simulink model "DRL_MPC_MATLAB"  (R2025a)
settings: Solver=FixedStepDiscrete  StartTime=0.0  StopTime=20  FixedStep=0.0005  RelTol=1e-3
PostLoadFcn:
  | addpath(fileparts(fileparts(get_param('DRL_MPC_MATLAB','FileName'))));setup_matlab_mpc;
undefined symbols (not defined in the file): controller_mode, mpc_initial_control_result, steering_interface_test, steering_test_deg
libraries: Solver_SF x1, rllib x1
settings Model: Creator=fengchengmin  LastModifiedBy=fengchengmin

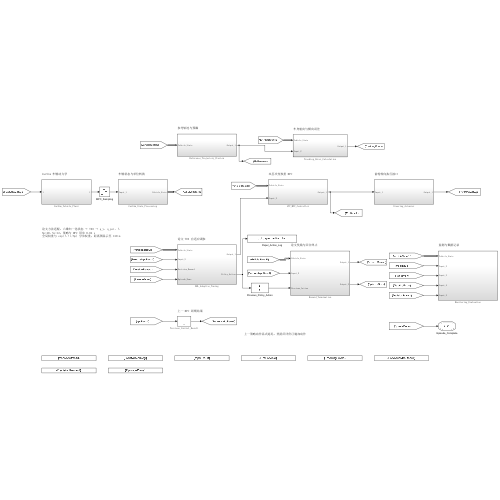
[thumbnail: Simulink's stored preview of the top-level diagram]
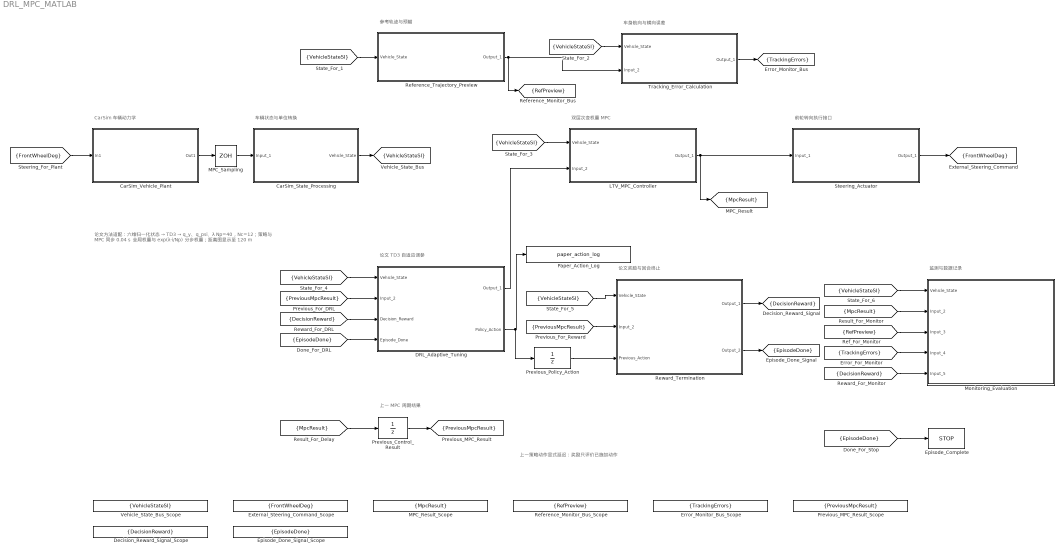
== system DRL_MPC_MATLAB ==
  note: 论文方法适配：六维归一化状态 → TD3 → q_y、q_psi、λ
      | Np=40，Nc=12；策略与 MPC 同步 0.04 s
      | 全局权重与 exp(λ·i/Np) 分步权重；距离图显示至 120 m
  note: 上一策略动作显式延迟：奖励只评价已施加动作
  note: CarSim 车辆动力学
  note: 车辆状态与单位转换
  note: 参考轨迹与预瞄
  note: 车身航向与横向误差
  note: 双层次变权重 MPC
  note: 论文 TD3 自适应调参
  note: 前轮转向执行接口
  note: 监测与数据记录
  note: 论文奖励与回合终止
  note: 上一 MPC 周期结果
  CarSim_State_Processing : Subsystem
  CarSim_Vehicle_Plant : Subsystem
  DRL_Adaptive_Tuning : Subsystem
  Decision_Reward_Signal_Scope : GotoTagVisibility  GotoTag=DecisionReward
  Episode_Complete : Stop
  Episode_Done_Signal_Scope : GotoTagVisibility  GotoTag=EpisodeDone
  Error_Monitor_Bus_Scope : GotoTagVisibility  GotoTag=TrackingErrors
  External_Steering_Command_Scope : GotoTagVisibility  GotoTag=FrontWheelDeg
  LTV_MPC_Controller : Subsystem
  MPC_Result_Scope : GotoTagVisibility  GotoTag=MpcResult
  MPC_Sampling : ZeroOrderHold  SampleTime=0.04
  Monitoring_Evaluation : Subsystem
  Paper_Action_Log : ToWorkspace  VariableName=paper_action_log  SaveFormat=Timeseries  SampleTime=-1
  Previous_Control_Result : UnitDelay  InitialCondition=mpc_initial_control_result  SampleTime=0.04  HasFrameUpgradeWarning=on
  Previous_MPC_Result_Scope : GotoTagVisibility  GotoTag=PreviousMpcResult
  Previous_Policy_Action : UnitDelay  InitialCondition=zeros(3,1)  SampleTime=.04  HasFrameUpgradeWarning=on
  Reference_Monitor_Bus_Scope : GotoTagVisibility  GotoTag=RefPreview
  Reference_Trajectory_Preview : Subsystem
  Reward_Termination : Subsystem
  Steering_Actuator : Subsystem
  Tracking_Error_Calculation : Subsystem
  Vehicle_State_Bus_Scope : GotoTagVisibility  GotoTag=VehicleStateSI
  tag scope: DecisionReward=scoped, EpisodeDone=scoped, FrontWheelDeg=scoped, MpcResult=scoped, PreviousMpcResult=scoped, RefPreview=scoped, TrackingErrors=scoped, VehicleStateSI=scoped
  wires:
  Tracking_Error_Calculation/1(Output_1) -> [TrackingErrors]
  Previous_Control_Result/1 -> [PreviousMpcResult]
  Reward_Termination/1(Output_1) -> [DecisionReward]
  Reward_Termination/2(Output_2) -> [EpisodeDone]
  [RefPreview] -> Monitoring_Evaluation/3(Input_3)
  [TrackingErrors] -> Monitoring_Evaluation/4(Input_4)
  [DecisionReward] -> Monitoring_Evaluation/5(Input_5)
  [EpisodeDone] -> Episode_Complete/1
  Steering_Actuator/1(Output_1) -> [FrontWheelDeg]
  [VehicleStateSI] -> LTV_MPC_Controller/1(Vehicle_State)
  [VehicleStateSI] -> Monitoring_Evaluation/1(Vehicle_State)
  CarSim_State_Processing/1(Vehicle_State) -> [VehicleStateSI]
  [FrontWheelDeg] -> CarSim_Vehicle_Plant/1(In1)
  [MpcResult] -> Previous_Control_Result/1
  [MpcResult] -> Monitoring_Evaluation/2(Input_2)
  LTV_MPC_Controller/1(Output_1) -> [MpcResult], Steering_Actuator/1(Input_1)
  MPC_Sampling/1 -> CarSim_State_Processing/1(Input_1)
  CarSim_Vehicle_Plant/1(Out1) -> MPC_Sampling/1
  [PreviousMpcResult] -> Reward_Termination/2(Input_2)
  Reference_Trajectory_Preview/1(Output_1) -> [RefPreview], Tracking_Error_Calculation/2(Input_2)
  [PreviousMpcResult] -> DRL_Adaptive_Tuning/2(Input_2)
  [DecisionReward] -> DRL_Adaptive_Tuning/3(Decision_Reward)
  [EpisodeDone] -> DRL_Adaptive_Tuning/4(Episode_Done)
  [VehicleStateSI] -> Reference_Trajectory_Preview/1(Vehicle_State)
  [VehicleStateSI] -> Tracking_Error_Calculation/1(Vehicle_State)
  [VehicleStateSI] -> DRL_Adaptive_Tuning/1(Vehicle_State)
  [VehicleStateSI] -> Reward_Termination/1(Vehicle_State)
  DRL_Adaptive_Tuning/1(Output_1) -> LTV_MPC_Controller/2(Input_2)
  Previous_Policy_Action/1 -> Reward_Termination/3(Previous_Action)
  DRL_Adaptive_Tuning/2(Policy_Action) -> Previous_Policy_Action/1, Paper_Action_Log/1

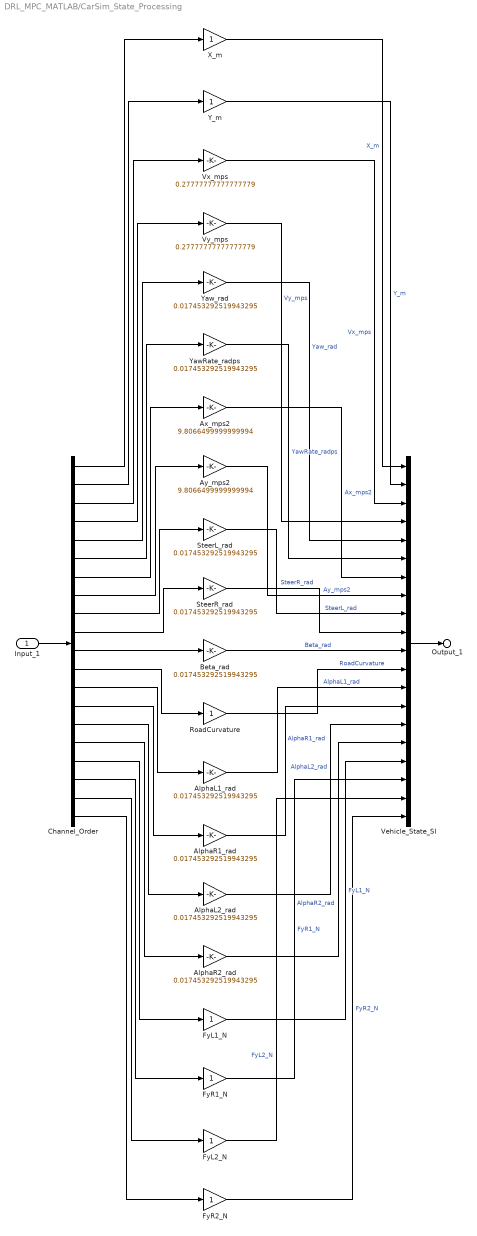
== system DRL_MPC_MATLAB/CarSim_State_Processing ==
  Input_1 : Inport
  AlphaL1_rad : Gain  Gain=0.017453292519943295
  AlphaL2_rad : Gain  Gain=0.017453292519943295
  AlphaR1_rad : Gain  Gain=0.017453292519943295
  AlphaR2_rad : Gain  Gain=0.017453292519943295
  Ax_mps2 : Gain  Gain=9.8066499999999994
  Ay_mps2 : Gain  Gain=9.8066499999999994
  Beta_rad : Gain  Gain=0.017453292519943295
  Channel_Order : Demux  Outputs=20
  FyL1_N : Gain
  FyL2_N : Gain
  FyR1_N : Gain
  FyR2_N : Gain
  RoadCurvature : Gain
  SteerL_rad : Gain  Gain=0.017453292519943295
  SteerR_rad : Gain  Gain=0.017453292519943295
  Vehicle_State_SI : BusCreator  Inputs=20
  Vx_mps : Gain  Gain=0.27777777777777779
  Vy_mps : Gain  Gain=0.27777777777777779
  X_m : Gain
  Y_m : Gain
  YawRate_radps : Gain  Gain=0.017453292519943295
  Yaw_rad : Gain  Gain=0.017453292519943295
  Output_1 : Outport  PortName=Vehicle_State
  wires:
  Vehicle_State_SI/1 -> Output_1/1
  FyR2_N/1 -> Vehicle_State_SI/20  "FyR2_N"
  Channel_Order/20 -> FyR2_N/1
  FyL2_N/1 -> Vehicle_State_SI/19  "FyL2_N"
  Channel_Order/19 -> FyL2_N/1
  FyR1_N/1 -> Vehicle_State_SI/18  "FyR1_N"
  Channel_Order/18 -> FyR1_N/1
  FyL1_N/1 -> Vehicle_State_SI/17  "FyL1_N"
  Channel_Order/17 -> FyL1_N/1
  AlphaR2_rad/1 -> Vehicle_State_SI/16  "AlphaR2_rad"
  Channel_Order/15 -> AlphaL2_rad/1
  Channel_Order/16 -> AlphaR2_rad/1
  AlphaL2_rad/1 -> Vehicle_State_SI/15  "AlphaL2_rad"
  AlphaR1_rad/1 -> Vehicle_State_SI/14  "AlphaR1_rad"
  Channel_Order/14 -> AlphaR1_rad/1
  AlphaL1_rad/1 -> Vehicle_State_SI/13  "AlphaL1_rad"
  Channel_Order/13 -> AlphaL1_rad/1
  RoadCurvature/1 -> Vehicle_State_SI/12  "RoadCurvature"
  Channel_Order/12 -> RoadCurvature/1
  Beta_rad/1 -> Vehicle_State_SI/11  "Beta_rad"
  Channel_Order/11 -> Beta_rad/1
  SteerR_rad/1 -> Vehicle_State_SI/10  "SteerR_rad"
  Channel_Order/10 -> SteerR_rad/1
  SteerL_rad/1 -> Vehicle_State_SI/9  "SteerL_rad"
  Channel_Order/9 -> SteerL_rad/1
  Ay_mps2/1 -> Vehicle_State_SI/8  "Ay_mps2"
  Channel_Order/8 -> Ay_mps2/1
  Ax_mps2/1 -> Vehicle_State_SI/7  "Ax_mps2"
  Channel_Order/7 -> Ax_mps2/1
  YawRate_radps/1 -> Vehicle_State_SI/6  "YawRate_radps"
  Channel_Order/6 -> YawRate_radps/1
  Yaw_rad/1 -> Vehicle_State_SI/5  "Yaw_rad"
  Channel_Order/5 -> Yaw_rad/1
  Vy_mps/1 -> Vehicle_State_SI/4  "Vy_mps"
  Channel_Order/4 -> Vy_mps/1
  Vx_mps/1 -> Vehicle_State_SI/3  "Vx_mps"
  Channel_Order/3 -> Vx_mps/1
  Y_m/1 -> Vehicle_State_SI/2  "Y_m"
  Channel_Order/2 -> Y_m/1
  X_m/1 -> Vehicle_State_SI/1  "X_m"
  Channel_Order/1 -> X_m/1
  Input_1/1 -> Channel_Order/1

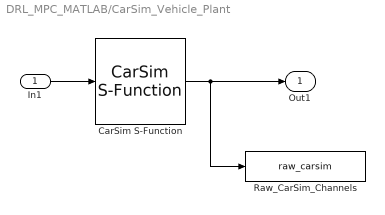
== system DRL_MPC_MATLAB/CarSim_Vehicle_Plant ==
  In1 : Inport
  CarSim S-Function : Solver_SF/CarSim S-Function  Priority=1  SIMFILE=C:\Users\fengchengmin\Desktop\JQRKZ\DRL-MPC\matlab\carsim\case\simfile.sim  Run_RTs=off  vs_state_ind=Run  StopMode_ind=Vehicle Model
  Raw_CarSim_Channels : ToWorkspace  VariableName=raw_carsim  SaveFormat=Timeseries  SampleTime=-1
  Out1 : Outport
  wires:
  CarSim S-Function/1 -> Out1/1, Raw_CarSim_Channels/1
  In1/1 -> CarSim S-Function/1

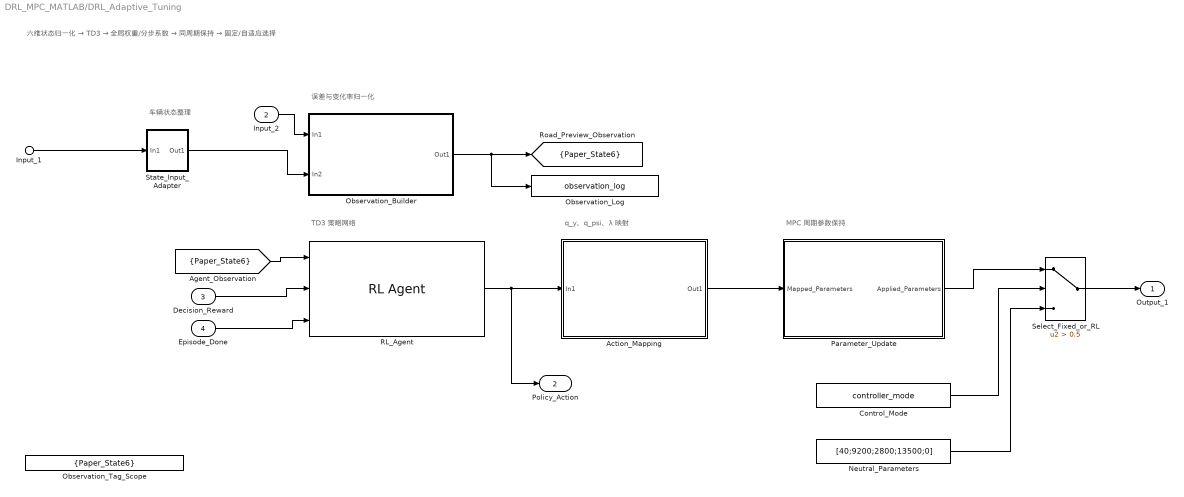
== system DRL_MPC_MATLAB/DRL_Adaptive_Tuning ==
  note: 六维状态归一化 → TD3 → 全局权重/分步系数 → 同周期保持 → 固定/自适应选择
  note: 车辆状态整理
  note: 误差与变化率归一化
  note: TD3 策略网络
  note: q_y、q_psi、λ 映射
  note: MPC 周期参数保持
  Input_1 : Inport  PortName=Vehicle_State
  Input_2 : Inport  Port=2
  Decision_Reward : Inport  Port=3
  Episode_Done : Inport  Port=4
  Action_Mapping : Subsystem
  Control_Mode : Constant  Value=controller_mode
  Neutral_Parameters : Constant  Value=[40;9200;2800;13500;0]
  Observation_Builder : Subsystem
  Observation_Log : ToWorkspace  VariableName=observation_log  SaveFormat=Timeseries  SampleTime=-1
  Observation_Tag_Scope : GotoTagVisibility  GotoTag=Paper_State6
  Parameter_Update : Subsystem
  RL_Agent : rllib/RL Agent  Agent=agent  ExternalActionAsInput=off  ProvideLastAction=off  ProvideCumRwd=off  TreatAsDirectFeedthrough=on  UseStrictObservationDataTypes=off
  Select_Fixed_or_RL : Switch  Criteria=u2 > Threshold  Threshold=0.5  SaturateOnIntegerOverflow=off  InputSameDT=off
  State_Input_Adapter : Subsystem
  Output_1 : Outport
  Policy_Action : Outport  Port=2
  tag scope: Paper_State6=scoped
  wires:
  Action_Mapping/1(Out1) -> Parameter_Update/1(Mapped_Parameters)
  Episode_Done/1 -> RL_Agent/3
  Decision_Reward/1 -> RL_Agent/2
  Input_2/1 -> Observation_Builder/1(In1)
  RL_Agent/1 -> Action_Mapping/1(In1), Policy_Action/1
  [Paper_State6] -> RL_Agent/1
  Select_Fixed_or_RL/1 -> Output_1/1
  Control_Mode/1 -> Select_Fixed_or_RL/2
  Neutral_Parameters/1 -> Select_Fixed_or_RL/3
  Observation_Builder/1(Out1) -> Observation_Log/1, [Paper_State6]
  Parameter_Update/1(Applied_Parameters) -> Select_Fixed_or_RL/1
  State_Input_Adapter/1(Out1) -> Observation_Builder/2(In2)
  Input_1/1 -> State_Input_Adapter/1(In1)

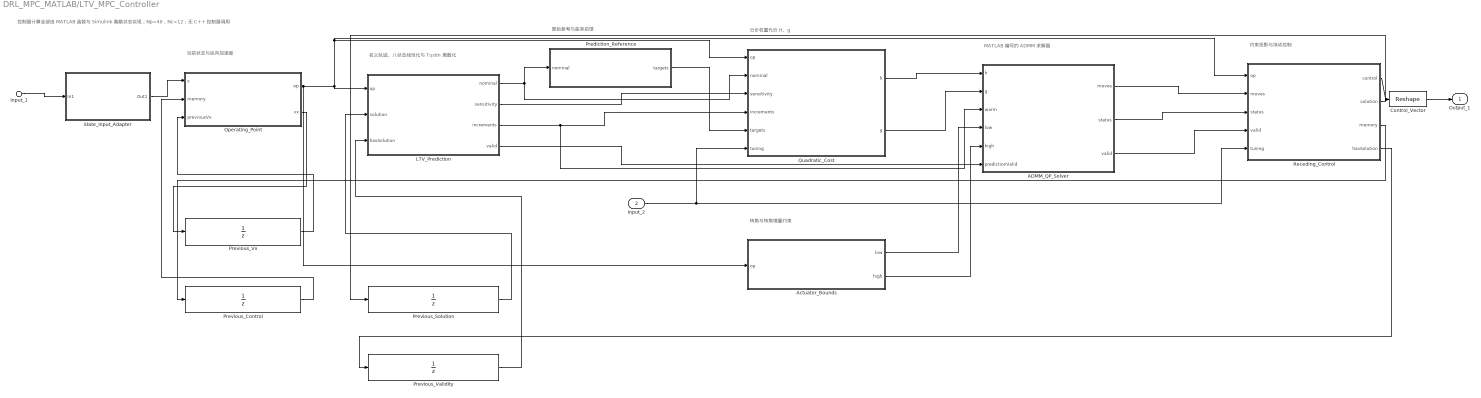
== system DRL_MPC_MATLAB/LTV_MPC_Controller ==
  note: 当前状态与纵向加速度
  note: 名义轨迹、八状态线性化与 Tustin 离散化
  note: 原始参考与曲率前馈
  note: 分步权重代价 H、g
  note: 转角与转角增量约束
  note: MATLAB 编写的 ADMM 求解器
  note: 约束投影与滚动控制
  note: 控制器计算全部由 MATLAB 函数与 Simulink 离散状态实现；Np=40，Nc=12；无 C++ 控制器调用
  Input_1 : Inport  PortName=Vehicle_State
  Input_2 : Inport  Port=2
  ADMM_QP_Solver : MATLAB Function  TreatAsAtomicUnit=on
  Actuator_Bounds : MATLAB Function  TreatAsAtomicUnit=on
  Control_Vector : Reshape
  LTV_Prediction : MATLAB Function  TreatAsAtomicUnit=on
  Operating_Point : MATLAB Function  TreatAsAtomicUnit=on
  Prediction_Reference : MATLAB Function  TreatAsAtomicUnit=on
  Previous_Control : UnitDelay  InitialCondition=[0;0]  SampleTime=.04  HasFrameUpgradeWarning=on
  Previous_Solution : UnitDelay  InitialCondition=zeros(12,1)  SampleTime=.04  HasFrameUpgradeWarning=on
  Previous_Validity : UnitDelay  InitialCondition=false  SampleTime=.04  HasFrameUpgradeWarning=on
  Previous_Vx : UnitDelay  InitialCondition=NaN  SampleTime=.04  HasFrameUpgradeWarning=on
  Quadratic_Cost : MATLAB Function  TreatAsAtomicUnit=on
  Receding_Control : MATLAB Function  TreatAsAtomicUnit=on
  State_Input_Adapter : Subsystem
  Output_1 : Outport
  wires:
  Input_1/1 -> State_Input_Adapter/1(In1)
  State_Input_Adapter/1(Out1) -> Operating_Point/1(s)
  Previous_Control/1 -> Operating_Point/2(memory)
  Previous_Vx/1 -> Operating_Point/3(previousVx)
  Operating_Point/2(vx) -> Previous_Vx/1
  Operating_Point/1(op) -> Quadratic_Cost/1(op), Receding_Control/1(op), LTV_Prediction/1(op), Actuator_Bounds/1(op)
  Previous_Solution/1 -> LTV_Prediction/2(solution)
  Previous_Validity/1 -> LTV_Prediction/3(hasSolution)
  LTV_Prediction/1(nominal) -> Prediction_Reference/1(nominal), Quadratic_Cost/2(nominal)
  LTV_Prediction/2(sensitivity) -> Quadratic_Cost/3(sensitivity)
  LTV_Prediction/3(increments) -> Quadratic_Cost/4(increments), ADMM_QP_Solver/3(warm)
  Prediction_Reference/1(targets) -> Quadratic_Cost/5(targets)
  Input_2/1 -> Quadratic_Cost/6(tuning), Receding_Control/5(tuning)
  Quadratic_Cost/1(h) -> ADMM_QP_Solver/1(h)
  Quadratic_Cost/2(g) -> ADMM_QP_Solver/2(g)
  Actuator_Bounds/1(low) -> ADMM_QP_Solver/4(low)
  Actuator_Bounds/2(high) -> ADMM_QP_Solver/5(high)
  LTV_Prediction/4(valid) -> ADMM_QP_Solver/6(predictionValid)
  ADMM_QP_Solver/1(moves) -> Receding_Control/2(moves)
  ADMM_QP_Solver/2(status) -> Receding_Control/3(status)
  ADMM_QP_Solver/3(valid) -> Receding_Control/4(valid)
  Receding_Control/1(control) -> Control_Vector/1
  Control_Vector/1 -> Output_1/1
  Receding_Control/2(solution) -> Previous_Solution/1
  Receding_Control/3(memory) -> Previous_Control/1
  Receding_Control/4(hasSolution) -> Previous_Validity/1

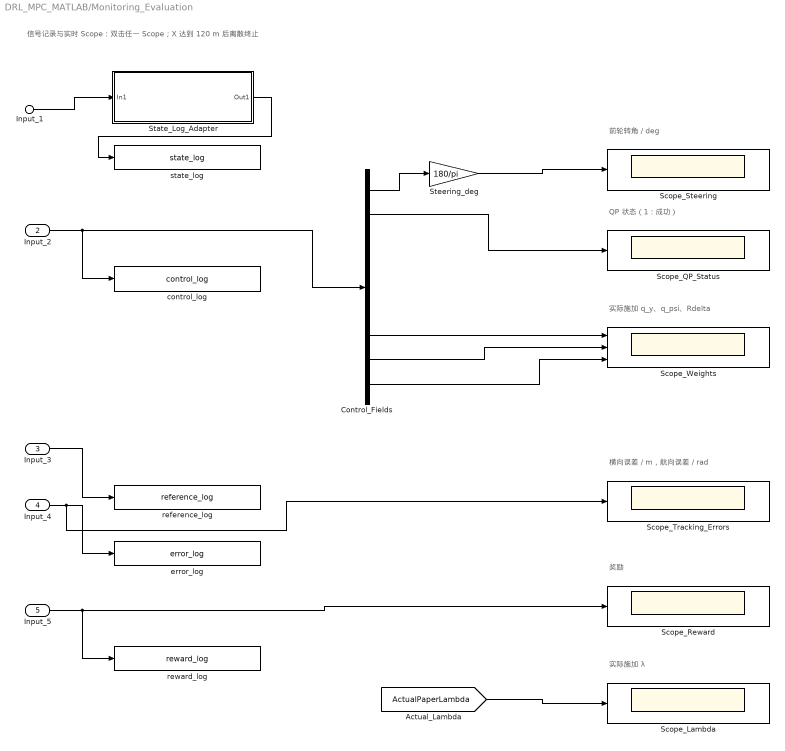
== system DRL_MPC_MATLAB/Monitoring_Evaluation ==
  note: 前轮转角 / deg
  note: QP 状态（1：成功）
  note: 实际施加 q_y、q_psi、Rdelta
  note: 横向误差 / m，航向误差 / rad
  note: 奖励
  note: 实际施加 λ
  note: 信号记录与实时 Scope：双击任一 Scope；X 达到 120 m 后离散终止
  Input_1 : Inport  PortName=Vehicle_State
  Input_2 : Inport  Port=2
  Input_3 : Inport  Port=3
  Input_4 : Inport  Port=4
  Input_5 : Inport  Port=5
  Control_Fields : Demux  Outputs=9
  Scope_Lambda : Scope
      settings: TimeSpan=8
  Scope_QP_Status : Scope
      settings: TimeSpan=8
  Scope_Reward : Scope
      settings: TimeSpan=8
  Scope_Steering : Scope
      settings: TimeSpan=8
  Scope_Tracking_Errors : Scope
      settings: TimeSpan=8
  Scope_Weights : Scope  NumInputPorts=3
      settings: TimeSpan=8
  State_Log_Adapter : Subsystem
  Steering_deg : Gain  Gain=180/pi
  control_log : ToWorkspace  VariableName=control_log  SaveFormat=Timeseries  SampleTime=-1
  error_log : ToWorkspace  VariableName=error_log  SaveFormat=Timeseries  SampleTime=-1
  reference_log : ToWorkspace  VariableName=reference_log  SaveFormat=Timeseries  SampleTime=-1
  reward_log : ToWorkspace  VariableName=reward_log  SaveFormat=Timeseries  SampleTime=-1
  state_log : ToWorkspace  VariableName=state_log  SaveFormat=Timeseries  SampleTime=-1
  wires:
  Input_5/1 -> reward_log/1, Scope_Reward/1
  Input_4/1 -> error_log/1, Scope_Tracking_Errors/1
  Input_3/1 -> reference_log/1
  Input_2/1 -> control_log/1, Control_Fields/1
  Control_Fields/1 -> Steering_deg/1
  Steering_deg/1 -> Scope_Steering/1
  Control_Fields/7 -> Scope_Weights/1
  Control_Fields/8 -> Scope_Weights/2
  Control_Fields/9 -> Scope_Weights/3
  Control_Fields/2 -> Scope_QP_Status/1
  [ActualPaperLambda] -> Scope_Lambda/1
  Input_1/1 -> State_Log_Adapter/1(In1)
  State_Log_Adapter/1(Out1) -> state_log/1

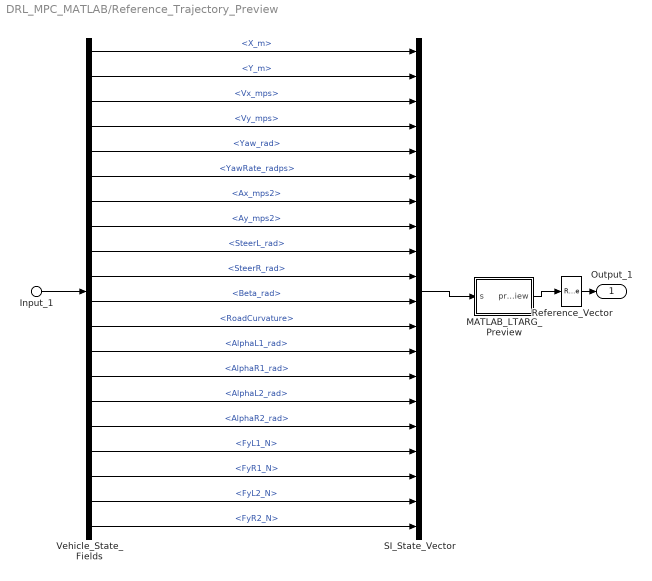
== system DRL_MPC_MATLAB/Reference_Trajectory_Preview ==
  Input_1 : Inport  PortName=Vehicle_State
  MATLAB_LTARG_Preview : MATLAB Function  TreatAsAtomicUnit=on
  Reference_Vector : Reshape
  SI_State_Vector : Mux  Inputs=20
  Vehicle_State_Fields : BusSelector  OutputSignals=X_m,Y_m,Vx_mps,Vy_mps,Yaw_rad,YawRate_radps,Ax_mps2,Ay_mps2,SteerL_rad,SteerR_rad,Beta_rad,RoadCurvature,AlphaL1_rad,AlphaR1_rad,AlphaL2_rad,AlphaR2_rad,FyL1_N,FyR1_N,FyL2_N,FyR2_N
  Output_1 : Outport
  wires:
  Input_1/1 -> Vehicle_State_Fields/1
  Vehicle_State_Fields/4 -> SI_State_Vector/4  "<Vy_mps>"
  Vehicle_State_Fields/5 -> SI_State_Vector/5  "<Yaw_rad>"
  Vehicle_State_Fields/20 -> SI_State_Vector/20  "<FyR2_N>"
  Vehicle_State_Fields/19 -> SI_State_Vector/19  "<FyL2_N>"
  Vehicle_State_Fields/18 -> SI_State_Vector/18  "<FyR1_N>"
  Vehicle_State_Fields/17 -> SI_State_Vector/17  "<FyL1_N>"
  Vehicle_State_Fields/16 -> SI_State_Vector/16  "<AlphaR2_rad>"
  Vehicle_State_Fields/15 -> SI_State_Vector/15  "<AlphaL2_rad>"
  Vehicle_State_Fields/14 -> SI_State_Vector/14  "<AlphaR1_rad>"
  Vehicle_State_Fields/13 -> SI_State_Vector/13  "<AlphaL1_rad>"
  Vehicle_State_Fields/12 -> SI_State_Vector/12  "<RoadCurvature>"
  Vehicle_State_Fields/11 -> SI_State_Vector/11  "<Beta_rad>"
  Vehicle_State_Fields/10 -> SI_State_Vector/10  "<SteerR_rad>"
  Vehicle_State_Fields/9 -> SI_State_Vector/9  "<SteerL_rad>"
  Vehicle_State_Fields/8 -> SI_State_Vector/8  "<Ay_mps2>"
  Vehicle_State_Fields/7 -> SI_State_Vector/7  "<Ax_mps2>"
  Vehicle_State_Fields/6 -> SI_State_Vector/6  "<YawRate_radps>"
  Vehicle_State_Fields/3 -> SI_State_Vector/3  "<Vx_mps>"
  Vehicle_State_Fields/2 -> SI_State_Vector/2  "<Y_m>"
  Vehicle_State_Fields/1 -> SI_State_Vector/1  "<X_m>"
  SI_State_Vector/1 -> MATLAB_LTARG_Preview/1(s)
  MATLAB_LTARG_Preview/1(preview) -> Reference_Vector/1
  Reference_Vector/1 -> Output_1/1

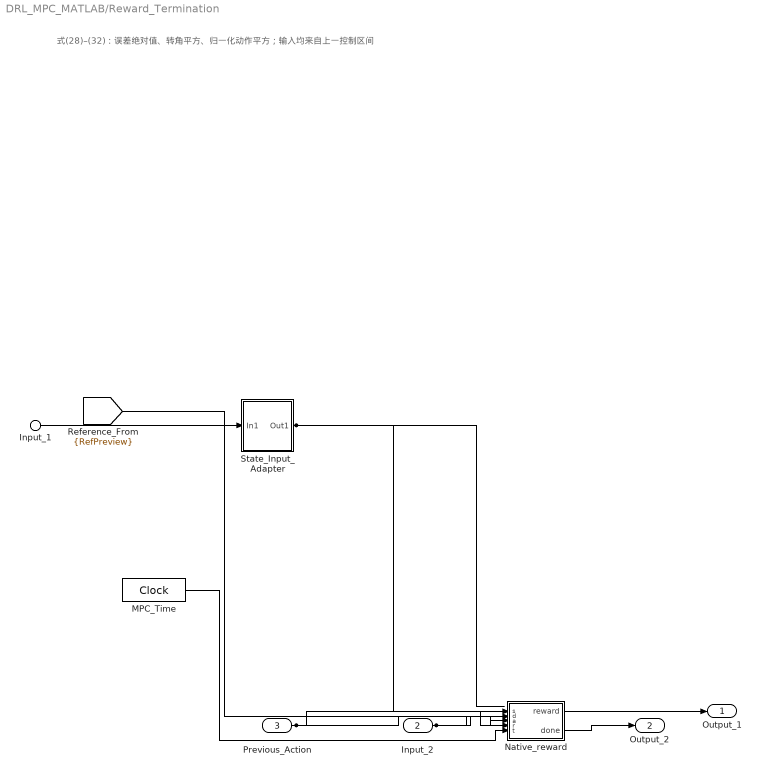
== system DRL_MPC_MATLAB/Reward_Termination ==
  note: 式(28)–(32)：误差绝对值、转角平方、归一化动作平方；输入均来自上一控制区间
  Input_1 : Inport  PortName=Vehicle_State
  Input_2 : Inport  Port=2
  Previous_Action : Inport  Port=3
  MPC_Time : DigitalClock  SampleTime=.04
  Native_reward : MATLAB Function  TreatAsAtomicUnit=on
  State_Input_Adapter : Subsystem
  Output_1 : Outport
  Output_2 : Outport  Port=2
  wires:
  Input_2/1 -> Native_reward/2(d)
  Previous_Action/1 -> Native_reward/3(a)
  State_Input_Adapter/1(Out1) -> Native_reward/1(s)
  Input_1/1 -> State_Input_Adapter/1(In1)
  [RefPreview] -> Native_reward/4(r)
  MPC_Time/1 -> Native_reward/5(t)
  Native_reward/1(reward) -> Output_1/1
  Native_reward/2(done) -> Output_2/1

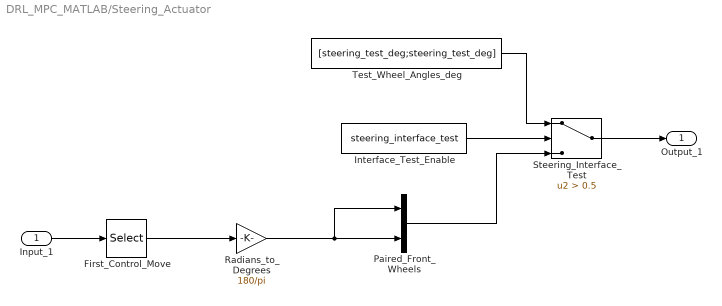
== system DRL_MPC_MATLAB/Steering_Actuator ==
  Input_1 : Inport
  First_Control_Move : Selector  InputPortWidth=9  IndexOptions=Index vector (dialog)  Indices=1  OutputSizes=1
  Interface_Test_Enable : Constant  Value=steering_interface_test
  Paired_Front_Wheels : Mux  Inputs=2
  Radians_to_Degrees : Gain  Gain=180/pi
  Steering_Interface_Test : Switch  Criteria=u2 > Threshold  Threshold=0.5  SaturateOnIntegerOverflow=off  InputSameDT=off
  Test_Wheel_Angles_deg : Constant  Value=[steering_test_deg;steering_test_deg]
  Output_1 : Outport
  wires:
  Paired_Front_Wheels/1 -> Steering_Interface_Test/3
  Test_Wheel_Angles_deg/1 -> Steering_Interface_Test/1
  Interface_Test_Enable/1 -> Steering_Interface_Test/2
  Steering_Interface_Test/1 -> Output_1/1
  Radians_to_Degrees/1 -> Paired_Front_Wheels/2, Paired_Front_Wheels/1
  First_Control_Move/1 -> Radians_to_Degrees/1
  Input_1/1 -> First_Control_Move/1

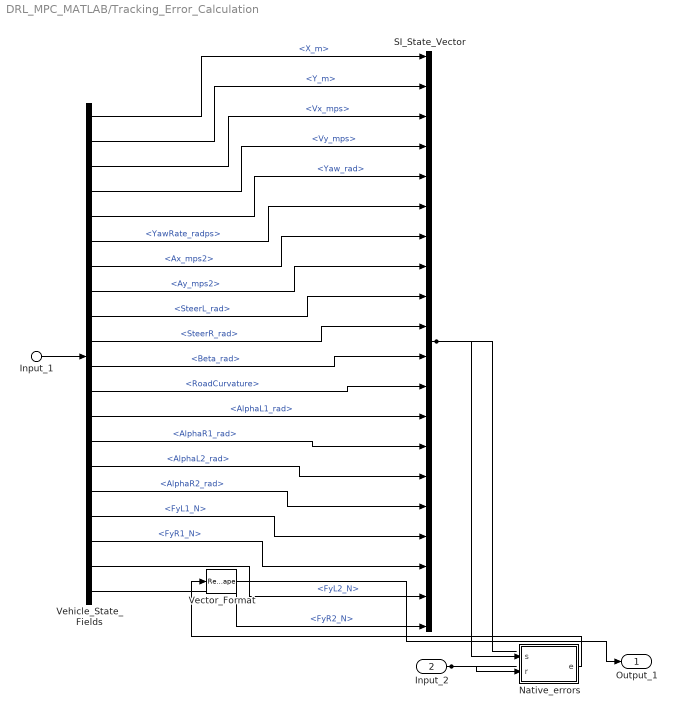
== system DRL_MPC_MATLAB/Tracking_Error_Calculation ==
  Input_1 : Inport  PortName=Vehicle_State
  Input_2 : Inport  Port=2
  Native_errors : MATLAB Function  TreatAsAtomicUnit=on
  SI_State_Vector : Mux  Inputs=20
  Vector_Format : Reshape
  Vehicle_State_Fields : BusSelector  OutputSignals=X_m,Y_m,Vx_mps,Vy_mps,Yaw_rad,YawRate_radps,Ax_mps2,Ay_mps2,SteerL_rad,SteerR_rad,Beta_rad,RoadCurvature,AlphaL1_rad,AlphaR1_rad,AlphaL2_rad,AlphaR2_rad,FyL1_N,FyR1_N,FyL2_N,FyR2_N
  Output_1 : Outport
  wires:
  Input_1/1 -> Vehicle_State_Fields/1
  Input_2/1 -> Native_errors/2(r)
  Vehicle_State_Fields/17 -> SI_State_Vector/17  "<FyL1_N>"
  SI_State_Vector/1 -> Native_errors/1(s)
  Vehicle_State_Fields/4 -> SI_State_Vector/4  "<Vy_mps>"
  Vehicle_State_Fields/5 -> SI_State_Vector/5  "<Yaw_rad>"
  Vehicle_State_Fields/20 -> SI_State_Vector/20  "<FyR2_N>"
  Vehicle_State_Fields/19 -> SI_State_Vector/19  "<FyL2_N>"
  Vehicle_State_Fields/18 -> SI_State_Vector/18  "<FyR1_N>"
  Vehicle_State_Fields/16 -> SI_State_Vector/16  "<AlphaR2_rad>"
  Vehicle_State_Fields/15 -> SI_State_Vector/15  "<AlphaL2_rad>"
  Vehicle_State_Fields/14 -> SI_State_Vector/14  "<AlphaR1_rad>"
  Vehicle_State_Fields/13 -> SI_State_Vector/13  "<AlphaL1_rad>"
  Vehicle_State_Fields/12 -> SI_State_Vector/12  "<RoadCurvature>"
  Vehicle_State_Fields/11 -> SI_State_Vector/11  "<Beta_rad>"
  Vehicle_State_Fields/10 -> SI_State_Vector/10  "<SteerR_rad>"
  Vehicle_State_Fields/9 -> SI_State_Vector/9  "<SteerL_rad>"
  Vehicle_State_Fields/8 -> SI_State_Vector/8  "<Ay_mps2>"
  Vehicle_State_Fields/7 -> SI_State_Vector/7  "<Ax_mps2>"
  Vehicle_State_Fields/6 -> SI_State_Vector/6  "<YawRate_radps>"
  Vehicle_State_Fields/3 -> SI_State_Vector/3  "<Vx_mps>"
  Vehicle_State_Fields/2 -> SI_State_Vector/2  "<Y_m>"
  Vehicle_State_Fields/1 -> SI_State_Vector/1  "<X_m>"
  Native_errors/1(e) -> Vector_Format/1
  Vector_Format/1 -> Output_1/1

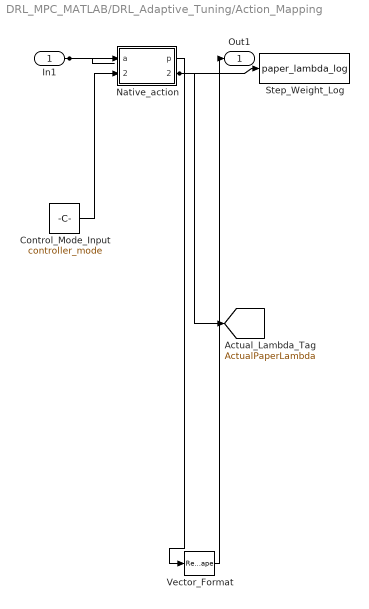
== system DRL_MPC_MATLAB/DRL_Adaptive_Tuning/Action_Mapping ==
  In1 : Inport
  Control_Mode_Input : Constant  Value=controller_mode
  Native_action : MATLAB Function  TreatAsAtomicUnit=on
  Step_Weight_Log : ToWorkspace  VariableName=paper_lambda_log  SaveFormat=Timeseries  SampleTime=-1
  Vector_Format : Reshape
  Out1 : Outport
  tag scope: ActualPaperLambda=global
  wires:
  In1/1 -> Native_action/1(a)
  Control_Mode_Input/1 -> Native_action/2(mode)
  Native_action/1(p) -> Vector_Format/1
  Vector_Format/1 -> Out1/1
  Native_action/2(lambda) -> Step_Weight_Log/1, [ActualPaperLambda]

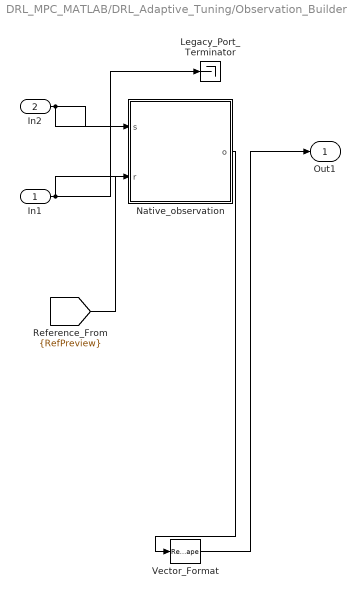
== system DRL_MPC_MATLAB/DRL_Adaptive_Tuning/Observation_Builder ==
  In1 : Inport
  In2 : Inport  Port=2
  Legacy_Port_Terminator : Terminator
  Native_observation : MATLAB Function  TreatAsAtomicUnit=on
  Vector_Format : Reshape
  Out1 : Outport
  wires:
  In1/1 -> Legacy_Port_Terminator/1
  In2/1 -> Native_observation/1(s)
  [RefPreview] -> Native_observation/2(r)
  Native_observation/1(o) -> Vector_Format/1
  Vector_Format/1 -> Out1/1

== system DRL_MPC_MATLAB/DRL_Adaptive_Tuning/Parameter_Update ==
  Mapped_Parameters : Inport
  MPC_Rate_Parameter_Hold : ZeroOrderHold  SampleTime=.04
  Applied_Parameters : Outport
  wires:
  MPC_Rate_Parameter_Hold/1 -> Applied_Parameters/1
  Mapped_Parameters/1 -> MPC_Rate_Parameter_Hold/1

== system DRL_MPC_MATLAB/DRL_Adaptive_Tuning/State_Input_Adapter ==
  In1 : Inport
  SI_State_Vector : Mux  Inputs=20
  Vehicle_State_Fields : BusSelector  OutputSignals=X_m,Y_m,Vx_mps,Vy_mps,Yaw_rad,YawRate_radps,Ax_mps2,Ay_mps2,SteerL_rad,SteerR_rad,Beta_rad,RoadCurvature,AlphaL1_rad,AlphaR1_rad,AlphaL2_rad,AlphaR2_rad,FyL1_N,FyR1_N,FyL2_N,FyR2_N
  Out1 : Outport
  wires:
  Vehicle_State_Fields/19 -> SI_State_Vector/19  "<FyL2_N>"
  Vehicle_State_Fields/13 -> SI_State_Vector/13  "<AlphaL1_rad>"
  Vehicle_State_Fields/8 -> SI_State_Vector/8  "<Ay_mps2>"
  Vehicle_State_Fields/10 -> SI_State_Vector/10  "<SteerR_rad>"
  Vehicle_State_Fields/20 -> SI_State_Vector/20  "<FyR2_N>"
  Vehicle_State_Fields/14 -> SI_State_Vector/14  "<AlphaR1_rad>"
  Vehicle_State_Fields/4 -> SI_State_Vector/4  "<Vy_mps>"
  Vehicle_State_Fields/16 -> SI_State_Vector/16  "<AlphaR2_rad>"
  Vehicle_State_Fields/2 -> SI_State_Vector/2  "<Y_m>"
  Vehicle_State_Fields/3 -> SI_State_Vector/3  "<Vx_mps>"
  Vehicle_State_Fields/18 -> SI_State_Vector/18  "<FyR1_N>"
  Vehicle_State_Fields/11 -> SI_State_Vector/11  "<Beta_rad>"
  Vehicle_State_Fields/15 -> SI_State_Vector/15  "<AlphaL2_rad>"
  Vehicle_State_Fields/5 -> SI_State_Vector/5  "<Yaw_rad>"
  Vehicle_State_Fields/12 -> SI_State_Vector/12  "<RoadCurvature>"
  Vehicle_State_Fields/17 -> SI_State_Vector/17  "<FyL1_N>"
  Vehicle_State_Fields/1 -> SI_State_Vector/1  "<X_m>"
  Vehicle_State_Fields/9 -> SI_State_Vector/9  "<SteerL_rad>"
  Vehicle_State_Fields/6 -> SI_State_Vector/6  "<YawRate_radps>"
  Vehicle_State_Fields/7 -> SI_State_Vector/7  "<Ax_mps2>"
  In1/1 -> Vehicle_State_Fields/1
  SI_State_Vector/1 -> Out1/1

== system DRL_MPC_MATLAB/LTV_MPC_Controller/State_Input_Adapter ==
  In1 : Inport
  SI_State_Vector : Mux  Inputs=20
  Vehicle_State_Fields : BusSelector  OutputSignals=X_m,Y_m,Vx_mps,Vy_mps,Yaw_rad,YawRate_radps,Ax_mps2,Ay_mps2,SteerL_rad,SteerR_rad,Beta_rad,RoadCurvature,AlphaL1_rad,AlphaR1_rad,AlphaL2_rad,AlphaR2_rad,FyL1_N,FyR1_N,FyL2_N,FyR2_N
  Out1 : Outport
  wires:
  Vehicle_State_Fields/5 -> SI_State_Vector/5  "<Yaw_rad>"
  Vehicle_State_Fields/18 -> SI_State_Vector/18  "<FyR1_N>"
  Vehicle_State_Fields/9 -> SI_State_Vector/9  "<SteerL_rad>"
  Vehicle_State_Fields/7 -> SI_State_Vector/7  "<Ax_mps2>"
  Vehicle_State_Fields/11 -> SI_State_Vector/11  "<Beta_rad>"
  Vehicle_State_Fields/8 -> SI_State_Vector/8  "<Ay_mps2>"
  Vehicle_State_Fields/10 -> SI_State_Vector/10  "<SteerR_rad>"
  Vehicle_State_Fields/3 -> SI_State_Vector/3  "<Vx_mps>"
  Vehicle_State_Fields/20 -> SI_State_Vector/20  "<FyR2_N>"
  Vehicle_State_Fields/15 -> SI_State_Vector/15  "<AlphaL2_rad>"
  Vehicle_State_Fields/4 -> SI_State_Vector/4  "<Vy_mps>"
  Vehicle_State_Fields/16 -> SI_State_Vector/16  "<AlphaR2_rad>"
  Vehicle_State_Fields/14 -> SI_State_Vector/14  "<AlphaR1_rad>"
  Vehicle_State_Fields/12 -> SI_State_Vector/12  "<RoadCurvature>"
  Vehicle_State_Fields/2 -> SI_State_Vector/2  "<Y_m>"
  Vehicle_State_Fields/6 -> SI_State_Vector/6  "<YawRate_radps>"
  Vehicle_State_Fields/13 -> SI_State_Vector/13  "<AlphaL1_rad>"
  Vehicle_State_Fields/19 -> SI_State_Vector/19  "<FyL2_N>"
  Vehicle_State_Fields/1 -> SI_State_Vector/1  "<X_m>"
  Vehicle_State_Fields/17 -> SI_State_Vector/17  "<FyL1_N>"
  In1/1 -> Vehicle_State_Fields/1
  SI_State_Vector/1 -> Out1/1

== system DRL_MPC_MATLAB/Monitoring_Evaluation/State_Log_Adapter ==
  In1 : Inport
  SI_State_Vector : Mux  Inputs=20
  Vehicle_State_Fields : BusSelector  OutputSignals=X_m,Y_m,Vx_mps,Vy_mps,Yaw_rad,YawRate_radps,Ax_mps2,Ay_mps2,SteerL_rad,SteerR_rad,Beta_rad,RoadCurvature,AlphaL1_rad,AlphaR1_rad,AlphaL2_rad,AlphaR2_rad,FyL1_N,FyR1_N,FyL2_N,FyR2_N
  Out1 : Outport
  wires:
  Vehicle_State_Fields/4 -> SI_State_Vector/4  "<Vy_mps>"
  Vehicle_State_Fields/3 -> SI_State_Vector/3  "<Vx_mps>"
  Vehicle_State_Fields/10 -> SI_State_Vector/10  "<SteerR_rad>"
  Vehicle_State_Fields/12 -> SI_State_Vector/12  "<RoadCurvature>"
  Vehicle_State_Fields/2 -> SI_State_Vector/2  "<Y_m>"
  Vehicle_State_Fields/6 -> SI_State_Vector/6  "<YawRate_radps>"
  Vehicle_State_Fields/13 -> SI_State_Vector/13  "<AlphaL1_rad>"
  Vehicle_State_Fields/5 -> SI_State_Vector/5  "<Yaw_rad>"
  Vehicle_State_Fields/11 -> SI_State_Vector/11  "<Beta_rad>"
  Vehicle_State_Fields/7 -> SI_State_Vector/7  "<Ax_mps2>"
  Vehicle_State_Fields/16 -> SI_State_Vector/16  "<AlphaR2_rad>"
  Vehicle_State_Fields/14 -> SI_State_Vector/14  "<AlphaR1_rad>"
  Vehicle_State_Fields/18 -> SI_State_Vector/18  "<FyR1_N>"
  Vehicle_State_Fields/9 -> SI_State_Vector/9  "<SteerL_rad>"
  Vehicle_State_Fields/8 -> SI_State_Vector/8  "<Ay_mps2>"
  Vehicle_State_Fields/1 -> SI_State_Vector/1  "<X_m>"
  Vehicle_State_Fields/19 -> SI_State_Vector/19  "<FyL2_N>"
  Vehicle_State_Fields/15 -> SI_State_Vector/15  "<AlphaL2_rad>"
  Vehicle_State_Fields/20 -> SI_State_Vector/20  "<FyR2_N>"
  Vehicle_State_Fields/17 -> SI_State_Vector/17  "<FyL1_N>"
  In1/1 -> Vehicle_State_Fields/1
  SI_State_Vector/1 -> Out1/1

== system DRL_MPC_MATLAB/Reward_Termination/State_Input_Adapter ==
  In1 : Inport
  SI_State_Vector : Mux  Inputs=20
  Vehicle_State_Fields : BusSelector  OutputSignals=X_m,Y_m,Vx_mps,Vy_mps,Yaw_rad,YawRate_radps,Ax_mps2,Ay_mps2,SteerL_rad,SteerR_rad,Beta_rad,RoadCurvature,AlphaL1_rad,AlphaR1_rad,AlphaL2_rad,AlphaR2_rad,FyL1_N,FyR1_N,FyL2_N,FyR2_N
  Out1 : Outport
  wires:
  Vehicle_State_Fields/4 -> SI_State_Vector/4  "<Vy_mps>"
  Vehicle_State_Fields/13 -> SI_State_Vector/13  "<AlphaL1_rad>"
  Vehicle_State_Fields/12 -> SI_State_Vector/12  "<RoadCurvature>"
  Vehicle_State_Fields/10 -> SI_State_Vector/10  "<SteerR_rad>"
  Vehicle_State_Fields/6 -> SI_State_Vector/6  "<YawRate_radps>"
  Vehicle_State_Fields/11 -> SI_State_Vector/11  "<Beta_rad>"
  Vehicle_State_Fields/9 -> SI_State_Vector/9  "<SteerL_rad>"
  Vehicle_State_Fields/20 -> SI_State_Vector/20  "<FyR2_N>"
  Vehicle_State_Fields/7 -> SI_State_Vector/7  "<Ax_mps2>"
  Vehicle_State_Fields/3 -> SI_State_Vector/3  "<Vx_mps>"
  Vehicle_State_Fields/5 -> SI_State_Vector/5  "<Yaw_rad>"
  Vehicle_State_Fields/1 -> SI_State_Vector/1  "<X_m>"
  In1/1 -> Vehicle_State_Fields/1
  Vehicle_State_Fields/2 -> SI_State_Vector/2  "<Y_m>"
  Vehicle_State_Fields/19 -> SI_State_Vector/19  "<FyL2_N>"
  Vehicle_State_Fields/14 -> SI_State_Vector/14  "<AlphaR1_rad>"
  Vehicle_State_Fields/15 -> SI_State_Vector/15  "<AlphaL2_rad>"
  Vehicle_State_Fields/16 -> SI_State_Vector/16  "<AlphaR2_rad>"
  Vehicle_State_Fields/17 -> SI_State_Vector/17  "<FyL1_N>"
  Vehicle_State_Fields/18 -> SI_State_Vector/18  "<FyR1_N>"
  Vehicle_State_Fields/8 -> SI_State_Vector/8  "<Ay_mps2>"
  SI_State_Vector/1 -> Out1/1

== matlab function DRL_MPC_MATLAB/LTV_MPC_Controller/ADMM_QP_Solver ==
  data: h input double size=[12 12]; moves output double size=[12 1]; g input double size=[12 1]; warm input double size=[12 1]; low input double size=[24 1]; high input double size=[24 1]; predictionValid input boolean size=1; status output double size=[4 1]; valid output boolean size=1; matlab_mpc_parameters parameter
function [moves,status,valid]=fcn(h,g,warm,low,high,predictionValid, matlab_mpc_parameters)
[moves,status,valid]=matlabAdmmQp(h,g,warm,low,high,matlab_mpc_parameters,predictionValid);
end

== matlab function DRL_MPC_MATLAB/LTV_MPC_Controller/Receding_Control ==
  data: op input double size=[13 1]; control output double size=[9 1]; moves input double size=[12 1]; status input double size=[4 1]; valid input boolean size=1; tuning input double size=[5 1]; solution output double size=[12 1]; memory output double size=[2 1]; hasSolution output boolean size=1; matlab_mpc_parameters parameter
function [control,solution,memory,hasSolution]=fcn(op,moves,status,valid,tuning, matlab_mpc_parameters)
[control,solution,memory,hasSolution]=matlabSteeringCommand(op,moves,status,valid,tuning,matlab_mpc_parameters);
end

== matlab function DRL_MPC_MATLAB/Reference_Trajectory_Preview/MATLAB_LTARG_Preview ==
  data: s input double size=[20 1]; preview output double size=[157 1]; matlab_mpc_parameters parameter
function preview=fcn(s, matlab_mpc_parameters)
preview=matlabReferencePreview(s,matlab_mpc_parameters);
end

== matlab function DRL_MPC_MATLAB/DRL_Adaptive_Tuning/Observation_Builder/Native_observation ==
  data: s input; o output; r input
function o=fcn(s,r)
ey=s(2)-r(1);ep=atan2(sin(s(5)-r(2)),cos(s(5)-r(2)));
xd=s(3)*cos(s(5))-s(4)*sin(s(5));yd=s(3)*sin(s(5))+s(4)*cos(s(5));
o=max(-1,min(1,[ey;ep;yd-r(4)*xd;s(6)-xd*r(3);s(3);r(3)]./[.25;.1;2;.5;30;.05]));
end

== matlab function DRL_MPC_MATLAB/Tracking_Error_Calculation/Native_errors ==
  data: s input; e output; r input
function e=fcn(s,r)
e=[s(2)-r(1);atan2(sin(s(5)-r(2)),cos(s(5)-r(2)))];
end

== matlab function DRL_MPC_MATLAB/DRL_Adaptive_Tuning/Action_Mapping/Native_action ==
  data: a input; p output; mode input; lambda output
function [p,lambda]=fcn(a,mode)
y=[25 55 85 115 155 200 240];h=[100 300 500 700 900 1000 1100 1300];l=[-1 -.7 -.5 -.3 0 .3 .5 1];
a=max(-1,min(1,a));lambda=l(1+round((a(3)+1)*3.5));
p=[40;80*y(1+round((a(1)+1)*3));4*h(1+round((a(2)+1)*3.5));13500;lambda];
if mode==2,lambda=0;p(5)=0;end
if mode==0,p=[40;9200;2800;13500;0];lambda=0;end
end

== matlab function DRL_MPC_MATLAB/Reward_Termination/Native_reward ==
  data: s input; reward output; d input; a input; r input; t input; done output
function [reward,done]=fcn(s,d,a,r,t)
ey=s(2)-r(1);ep=atan2(sin(s(5)-r(2)),cos(s(5)-r(2)));
reward=-300*abs(ey)/.25-50*abs(ep)/.1-60*d(1)^2-15*a(1)^2-15*a(2)^2-20*a(3)^2;
failed=any(~isfinite(s))||abs(ey)>1.5||abs(s(11))>8*pi/180;
done=double(failed||s(1)>=120||t>=19.999);if failed,reward=reward-100;end
end

== matlab function DRL_MPC_MATLAB/LTV_MPC_Controller/Operating_Point ==
  data: s input double size=[20 1]; op output double size=[13 1]; memory input double size=[2 1]; previousVx input double size=1; vx output double size=1
function [op,vx]=fcn(s,memory,previousVx)
op=matlabOperatingPoint(s,memory,previousVx);vx=s(3);
end

== matlab function DRL_MPC_MATLAB/LTV_MPC_Controller/LTV_Prediction ==
  data: op input double size=[13 1]; nominal output double size=[8 41]; solution input double size=[12 1]; hasSolution input boolean size=1; sensitivity output double size=[8 12 40]; increments output double size=[12 1]; valid output boolean size=1; matlab_mpc_parameters parameter
function [nominal,sensitivity,increments,valid]=fcn(op,solution,hasSolution, matlab_mpc_parameters)
[nominal,sensitivity,increments,valid]=matlabNominalPrediction(op,solution,hasSolution,matlab_mpc_parameters);
end

== matlab function DRL_MPC_MATLAB/LTV_MPC_Controller/Prediction_Reference ==
  data: nominal input double size=[8 41]; targets output double size=[9 40]; matlab_mpc_parameters parameter
function targets=fcn(nominal, matlab_mpc_parameters)
targets=matlabPredictionReference(nominal,matlab_mpc_parameters);
end

== matlab function DRL_MPC_MATLAB/LTV_MPC_Controller/Quadratic_Cost ==
  data: op input double size=[13 1]; h output double size=[12 12]; nominal input double size=[8 41]; sensitivity input double size=[8 12 40]; increments input double size=[12 1]; targets input double size=[9 40]; tuning input double size=[5 1]; g output double size=[12 1]; matlab_mpc_parameters parameter
function [h,g]=fcn(op,nominal,sensitivity,increments,targets,tuning, matlab_mpc_parameters)
[h,g]=matlabCostMatrices(op,nominal,sensitivity,increments,targets,tuning,matlab_mpc_parameters);
end

== matlab function DRL_MPC_MATLAB/LTV_MPC_Controller/Actuator_Bounds ==
  data: op input double size=[13 1]; low output double size=[24 1]; high output double size=[24 1]; matlab_mpc_parameters parameter
function [low,high]=fcn(op, matlab_mpc_parameters)
[low,high]=matlabConstraintBounds(op,matlab_mpc_parameters);
end
